simulink model "test_vcu128"  (R2018a)
settings: Solver=VariableStepDiscrete  StartTime=0.0  StopTime=10.0  RelTol=1e-3
libraries: xbsIndex_r4 x12, xps_library x2
settings Model: Creator=jackh  LastModifiedBy=hpw1
settings OptimizationCC: DefaultParameterBehavior=Inlined
settings CodeAppCC: StateflowObjectComments=on

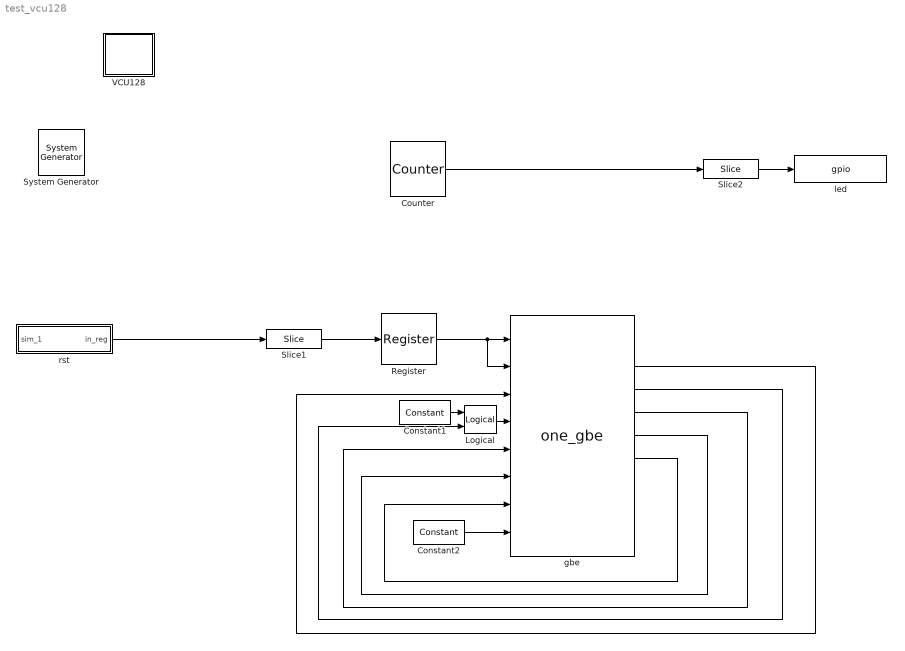
== system test_vcu128 ==
  " System Generator" : xbsIndex_r4/ System Generator  Tag=genX  xilinxfamily=virtexuplusHBM  part=xcvu37p  speed=-2L-e  package=fsvh2892  synthesis_tool=XST  clock_wrapper=Clock Enables  directory=/home/hpw1/amit/mlib_devel/test_vcu128/sysgen  proj_type=Vivado  Synth_file=Vivado Synthesis Defaults  Impl_file=Vivado Implementation Defaults  testbench=off  simulink_period=1  sysclk_period=10  dcm_input_clock_period=10  incr_netlist=off  trim_vbits=Everywhere in SubSystem  dbl_ovrd=According to Block Masks  core_generation=According to Block Masks  run_coregen=off  deprecated_control=off  eval_field=0  block_type=sysgen
  Constant1 : xbsIndex_r4/Constant  const=1  gui_display_data_type=Boolean  arith_type=Boolean  n_bits=32  bin_pt=0  preci_type=Single  exp_width=8  frac_width=24  explicit_period=on  period=1  equ=P=C  opselect=C  inp2=PCIN>>17  opr=+  inp1=P  carry=CIN  dbl_ovrd=off  block_type=constant
  Constant2 : xbsIndex_r4/Constant  const=1  gui_display_data_type=Boolean  arith_type=Boolean  n_bits=32  bin_pt=0  preci_type=Single  exp_width=8  frac_width=24  explicit_period=on  period=1  equ=P=C  opselect=C  inp2=PCIN>>17  opr=+  inp1=P  carry=CIN  dbl_ovrd=off  block_type=constant
  Counter : xbsIndex_r4/Counter  cnt_type=Free Running  cnt_to=Inf  operation=Up  start_count=0  cnt_by_val=1  arith_type=Unsigned  n_bits=32  bin_pt=0  load_pin=off  rst=off  en=off  explicit_period=on  period=1  use_behavioral_HDL=off  implementation=Fabric  dbl_ovrd=off  block_type=counter
  Logical : xbsIndex_r4/Logical  logical_function=AND  inputs=2  en=off  latency=0  precision=Full  arith_type=Unsigned  n_bits=16  bin_pt=0  align_bp=on  dbl_ovrd=off  block_type=logical
  Register : xbsIndex_r4/Register  init=0  rst=off  en=off  dbl_ovrd=off  block_type=register
  Slice1 : xbsIndex_r4/Slice  nbits=1  boolean_output=on  mode=Lower Bit Location + Width  bit1=0  base1=MSB of Input  bit0=0  base0=LSB of Input  dbl_ovrd=off  block_type=slice
  Slice2 : xbsIndex_r4/Slice  nbits=1  boolean_output=on  mode=Upper Bit Location + Width  bit1=-5  base1=MSB of Input  bit0=0  base0=LSB of Input  dbl_ovrd=off  block_type=slice
  VCU128 : Subsystem  Tag=xps:xsg  mask(xsg core config){hw_sys=VCU128:xcvu37p, clk_src=sys_clk, clk_rate=100, use_microblaze=on, sample_period=1, synthesis_tool=XST}
      mask prompts: hw_sys "Hardware Platform"; clk_src "User IP Clock source"; clk_rate "User IP Clock Rate (MHz)"; use_microblaze "Use Microblaze controller?"; sample_period "Sample Period"; synthesis_tool "Synthesis Tool:"
      mask help:
      | The XSG Core Config block is used to configure the System Generator design
      | for the casper_xps toolflow. Settings here are used to configure the
      | Xilinx System Generator block parameters automatically, and control toolflow
      | script  execution. It needs to be at the top level of all designs being compiled
      | with the casper_xps toolflow.
      mask init:
      | xps_xsg_vcu128_conf_mask;
      mask Help: eval('xlWeb([getenv(''MLIB_ROOT''), ''\doc\html\sys_xsg_core_config\sys_xsg_core_config.html''])')
      mask TypeOptions hw_sys: VCU128:xcvu37p
      mask TypeOptions clk_src: sys_clk
      mask TypeOptions synthesis_tool: Leonardo Spectrum | Synplify | Synplify Pro | XST
      mask Display: fprintf(['VCU128']);
  gbe : xps_library/IO/one_gbe  Tag=xps:onegbe  local_en=on  dis_cpu_rx=off  dis_cpu_tx=off  cpu_promiscuous=off  local_mac=hex2dec('123456789abc')  local_ip=hex2dec('c0a8290a')  local_port=4321  local_gateway=1
      settings: SourceProductName=CASPER XPS Blockset
  led : xps_library/IO/gpio  Tag=xps:gpio  io_group_params_forwarded=on  io_group=ROACH:led  io_group_real=led  io_group_custom=0  io_dir=out  arith_type=Boolean  bitwidth=1  bin_pt=0  bit_index=0  sample_period=1  use_single_ended=off  use_ddr=off  reg_iob=on  reg_clk_phase=0  termination=None
      settings: SourceProductName=CASPER XPS Blockset
  rst : Subsystem  Tag=xps:sw_reg  AncestorBlock=xps_library/Memory/software_register  mask(swreg){io_dir=From Processor, io_delay=0, init_val=0, sample_period=1, names=reg, bitwidths=32, bin_pts=0, arith_types=0, sim_port=on, show_format=on}
      mask prompts: io_dir "I/O direction"; io_delay "I/O delay"; init_val "Initial Value"; sample_period "Sample period"; names "Bitfield names [msb...lsb]"; bitwidths "Bitfield widths"; bin_pts "Bitfield binary pts"; arith_types "Bitfield types, ufix=0, fix=1, bool=2"; sim_port "Provide sim input/output?"; show_format "Print format string?"
      mask help: A 32-bit software-accessible register. Can be divided into bitfields of varying widths and types using the fields in the block mask.
      mask init:
      | swreg_init(gcb)
      settings: AttributesFormatString=1input:uf32.0 = 32 bits
      mask TypeOptions io_dir: To Processor | From Processor
      mask Callback io_dir:
      | mask_enables = get_param(gcb, 'MaskEnables');
      | mask_names = get_param(gcb, 'MaskNames');
      | if strcmp(get_param(gcb, 'io_dir'), 'To Processor'),
      |     mask_enables{ismember(mask_names, 'sample_period')} = 'off';
      | else
      |     mask_enables{ismember(mask_names, 'sample_period')} = 'on';
      | end
      | set_param(gcb, 'MaskEnables', mask_enables);
      mask DialogControl ParameterTabVar0 Prompt: Setup
  wires:
  Counter/1 -> Slice2/1
  Register/1 -> gbe/2, gbe/1
  Logical/1 -> gbe/4
  gbe/5 -> gbe/5
  gbe/6 -> gbe/6
  Constant2/1 -> gbe/8
  gbe/3 -> gbe/3
  gbe/7 -> gbe/7
  Slice1/1 -> Register/1
  rst/1(in_reg) -> Slice1/1
  Constant1/1 -> Logical/1
  gbe/4 -> Logical/2
  Slice2/1 -> led/1

== system test_vcu128/VCU128 ==

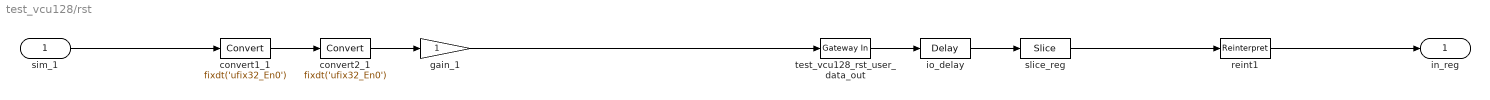
== system test_vcu128/rst ==
  sim_1 : Inport
  convert1_1 : DataTypeConversion  OutDataTypeStr=fixdt('ufix32_En0')  LockScale=on
  convert2_1 : DataTypeConversion  OutDataTypeStr=fixdt('ufix32_En0')  ConvertRealWorld=Stored Integer (SI)  LockScale=on
  gain_1 : Gain
  io_delay : xbsIndex_r4/Delay  rst=off  infoeditControl=Selection of Reset will increase slice count due to use of real FFs and instead of SRLs  en=off  latency=0  reg_retiming=on  dbl_ovrd=off  block_type=delay
  reint1 : xbsIndex_r4/Reinterpret  force_arith_type=on  arith_type=Unsigned  force_bin_pt=on  bin_pt=0  block_type=reinterpret
  slice_reg : xbsIndex_r4/Slice  nbits=32  boolean_output=off  mode=Lower Bit Location + Width  bit1=0  base1=MSB of Input  bit0=0  base0=LSB of Input  dbl_ovrd=off  block_type=slice
  test_vcu128_rst_user_data_out : xbsIndex_r4/Gateway In  gui_display_data_type=Fixed-point  arith_type=Unsigned  n_bits=32  bin_pt=0  preci_type=Single  exp_width=8  frac_width=24  rows=1  columns=1  quantization="Round  (unbiased: +/- Inf)"  overflow=Saturate  period=1  UseAsADC=off  ADCChannel='1'  interface=None  automatic_assignment=on  address_offset=hex2dec('00')  intf_name=''  intf_description=''  default_value=0  timing_constraint=None  locs_specified=off  LOCs={}  io_standard={}  inherit_from_input=off  hdl_port=on  dbl_ovrd=off  block_type=gatewayin
  in_reg : Outport
  wires:
  test_vcu128_rst_user_data_out/1 -> io_delay/1
  sim_1/1 -> convert1_1/1
  convert1_1/1 -> convert2_1/1
  convert2_1/1 -> gain_1/1
  gain_1/1 -> test_vcu128_rst_user_data_out/1
  io_delay/1 -> slice_reg/1
  slice_reg/1 -> reint1/1
  reint1/1 -> in_reg/1
